simulink model "Fault Response Project - Traffic Light"  (R2026a)
settings: Solver=VariableStepAuto  StopTime=60
StartFcn:
  | learning.simulink.modelCallbacks.startFunction(gcs);
StopFcn:
  | learning.simulink.modelCallbacks.stopFunction(gcs);
model workspace (MAT data in the model file):
  courseObject.course = 'stateflow'
  courseObject.chapter = 10
  courseObject.lesson = 1
  courseObject.section = 2
  courseObject.task = 1
libraries: SignalEditorBlockLib x1, signalChecks x1
CloseFcn:
  | learning.simulink.cleanupOnlineTraining;learning.simulink.Application.getInstance().dduxLogMatlabEvent("ModelClosed");
Description:
  | TrainingCourseModel
settings Model: Creator=PC  LastModifiedBy=PC

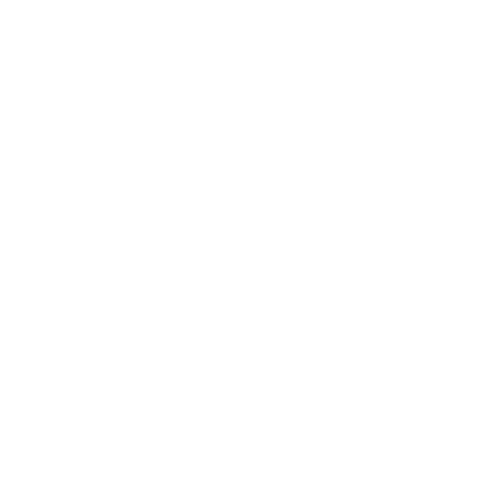
[thumbnail: Simulink's stored preview of the top-level diagram]
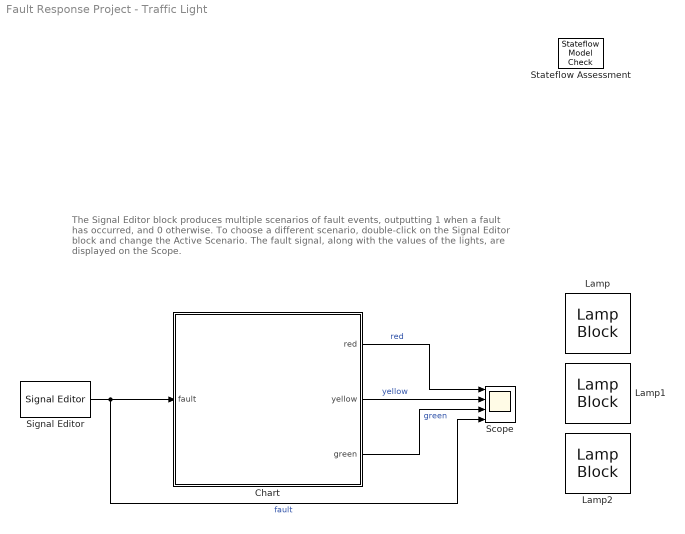
== system Fault Response Project - Traffic Light ==
  note: The Signal Editor block produces multiple scenarios of fault events, outputting 1 when a fault has occurred, and 0 otherwise.
      |
      | To choose a different scenario, double-click on the Signal Editor block and change the Active Scenario.
      |
      | The fault signal, along with the values of the lights, are displayed on the Scope.
  Chart : Stateflow chart  TreatAsAtomicUnit=on
  Lamp : LampBlock  LabelPosition=Hide  DefaultColor=[192.0, 192.0, 192.0]
  Lamp1 : LampBlock  LabelPosition=Hide  DefaultColor=[192.0, 192.0, 192.0]
  Lamp2 : LampBlock  LabelPosition=Hide  DefaultColor=[192.0, 192.0, 192.0]
  Scope : Scope  NumInputPorts=4
      settings: ActiveDisplayYMinimum=-0.12499999999999997  ActiveDisplayYMaximum=1.125
  Signal Editor : SignalEditorBlockLib/Signal Editor  FileName=trafficLightFault.mat  ActiveScenario=Faults  ActiveSignal=fault  IsBus=off  OutputBusObjectStr=Bus: BusObject  SampleTime=1  Interpolate=off  ZeroCross=off  OutputAfterFinalValue=Setting to zero  Unit=inherit  PreserveSignalName=on  ApplySigPropsToAllScenarios=on  ApplySigPropsToAllSignals=off  SignalPropertySource=Dialog parameters
  Stateflow Assessment : signalChecks/Stateflow Model Check  mlfunc='LearningApplication.gradeStateflowTask'  flags='conditionTransitions'  startInChart=true  lesson=0  task=6  pass=-1
      settings: AttributesFormatString=|
      | No input required
      | for this task
  wires:
  Signal Editor/1 -> Chart/1(fault), Scope/4  "fault"
  Chart/2(yellow) -> Scope/2  "yellow"
  Chart/3(green) -> Scope/3  "green"
  Chart/1(red) -> Scope/1  "red"

== stateflow chart Fault Response Project - Traffic Light/Chart ==
  state Normal
    state Stop
      entry:
      red = 1;
      yellow = 0;
      green = 0;
    state PrepareToStop
      entry:
      red = 0;
      yellow = 1;
      green = 0;
    state Go
      entry:
      red = 0;
      yellow = 0;
      green = 1;
    (default) -> Stop
    Stop -> (junction 26)
    (junction 26) -> (junction 29) : after(3,sec)
    PrepareToStop -> Stop : after(3,sec)
    Go -> PrepareToStop : after(10,sec)
    (junction 29) -> Go
  state Fault
    entry:
    yellow = 0;
    green = 0;
    state BlinkOn
      entry:
      red = 1;
    state BlinkOff
      entry:
      red = 0;
    (default) -> BlinkOn
    BlinkOn -> BlinkOff : after(1,sec)
    BlinkOff -> BlinkOn : after(1,sec)
  (default) -> Normal
  Normal -> Fault : [fault == 1]
  Fault -> Normal : [fault == 0]
  data: red output =1; yellow output; fault input; green output =0
